simulink subsystem "adaptiveEcm"  (R2025b)
settings: Solver=VariableStepAuto  StartTime=0.0  StopTime=10.0  RelTol=1e-3
values from neighbouring files (symbols this model uses):
  ECM = ecmParams(TempDep=false, Degradation=false, IC=struct("soc0", zD(1, :), "T0C", mean(tC(1, :))))    [checkFastPlant.m]
undefined symbols (not defined in the file or in its folder): diff, trace
(part 2 of 2)

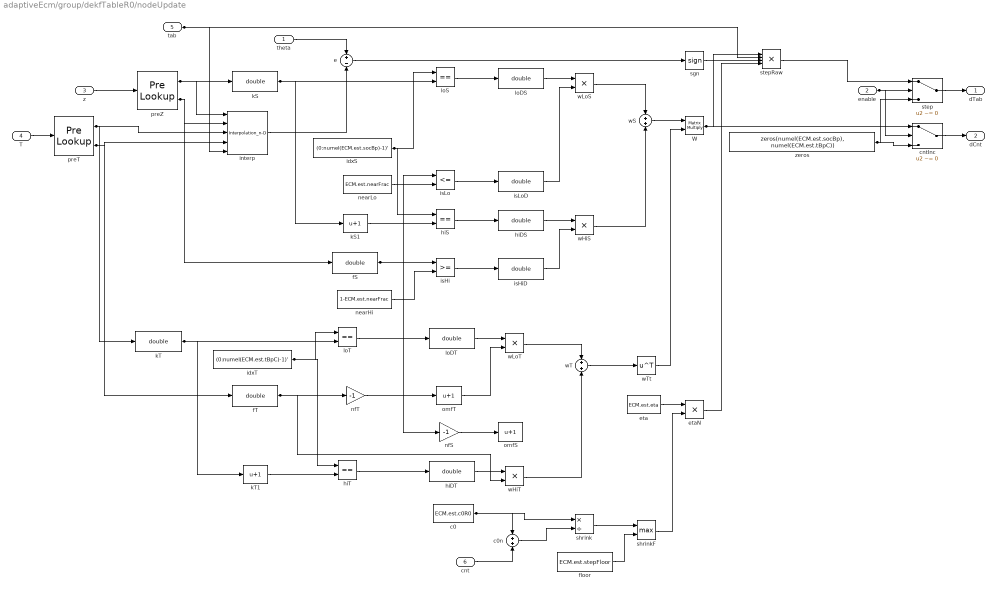
== system adaptiveEcm/group/dekfTableR0/nodeUpdate ==
  theta : Inport  PortDimensions=1
  enable : Inport  Port=2  PortDimensions=1
  z : Inport  Port=3  PortDimensions=1
  T : Inport  Port=4  PortDimensions=1
  tab : Inport  Port=5  PortDimensions=[numel(ECM.est.socBp) numel(ECM.est.tBpC)]
  cnt : Inport  Port=6  PortDimensions=[numel(ECM.est.socBp) numel(ECM.est.tBpC)]
  W : Product  Multiplication=Matrix(*)
  c0 : Constant  Value=ECM.est.c0R0
  c0n : Sum
  cntInc : Switch  Criteria=u2 ~= 0  SaturateOnIntegerOverflow=off  InputSameDT=off
  e : Sum  Inputs=+-
  eta : Constant  Value=ECM.est.eta
  etaN : Product
  fS : DataTypeConversion  OutDataTypeStr=double  SaturateOnIntegerOverflow=off  RndMeth=Floor
  fT : DataTypeConversion  OutDataTypeStr=double  SaturateOnIntegerOverflow=off  RndMeth=Floor
  floor : Constant  Value=ECM.est.stepFloor
  hiDS : DataTypeConversion  OutDataTypeStr=double  SaturateOnIntegerOverflow=off  RndMeth=Floor
  hiDT : DataTypeConversion  OutDataTypeStr=double  SaturateOnIntegerOverflow=off  RndMeth=Floor
  hiS : RelationalOperator  Operator===  OutDataTypeStr=boolean  RndMeth=Simplest  InputSameDT=off
  hiT : RelationalOperator  Operator===  OutDataTypeStr=boolean  RndMeth=Simplest  InputSameDT=off
  idxS : Constant  Value=(0:numel(ECM.est.socBp)-1)'
  idxT : Constant  Value=(0:numel(ECM.est.tBpC)-1)'
  interp : Interpolation_n-D  TableSource=Input port  InternalRulePriority=Speed
      settings: InputPortMap=u0,u1,u2,u3,p2
  isHi : RelationalOperator  OutDataTypeStr=boolean  RndMeth=Simplest  InputSameDT=off
  isHiD : DataTypeConversion  OutDataTypeStr=double  SaturateOnIntegerOverflow=off  RndMeth=Floor
  isLo : RelationalOperator  Operator=<=  OutDataTypeStr=boolean  RndMeth=Simplest  InputSameDT=off
  isLoD : DataTypeConversion  OutDataTypeStr=double  SaturateOnIntegerOverflow=off  RndMeth=Floor
  kS : DataTypeConversion  OutDataTypeStr=double  SaturateOnIntegerOverflow=off  RndMeth=Floor
  kS1 : Bias  Bias=1  SaturateOnIntegerOverflow=off
  kT : DataTypeConversion  OutDataTypeStr=double  SaturateOnIntegerOverflow=off  RndMeth=Floor
  kT1 : Bias  Bias=1  SaturateOnIntegerOverflow=off
  loDS : DataTypeConversion  OutDataTypeStr=double  SaturateOnIntegerOverflow=off  RndMeth=Floor
  loDT : DataTypeConversion  OutDataTypeStr=double  SaturateOnIntegerOverflow=off  RndMeth=Floor
  loS : RelationalOperator  Operator===  OutDataTypeStr=boolean  RndMeth=Simplest  InputSameDT=off
  loT : RelationalOperator  Operator===  OutDataTypeStr=boolean  RndMeth=Simplest  InputSameDT=off
  nearHi : Constant  Value=1-ECM.est.nearFrac
  nearLo : Constant  Value=ECM.est.nearFrac
  nfS : Gain  Gain=-1
  nfT : Gain  Gain=-1
  omfS : Bias  Bias=1  SaturateOnIntegerOverflow=off
  omfT : Bias  Bias=1  SaturateOnIntegerOverflow=off
  preT : PreLookup  BreakpointsData=ECM.est.tBpC
  preZ : PreLookup  BreakpointsData=ECM.est.socBp
  sgn : Signum
  shrink : Product  Inputs=*/
  shrinkF : MinMax  Function=max  Inputs=2
  step : Switch  Criteria=u2 ~= 0  SaturateOnIntegerOverflow=off  InputSameDT=off
  stepRaw : Product  Inputs=4
  wHiS : Product
  wHiT : Product
  wLoS : Product
  wLoT : Product
  wS : Sum
  wT : Sum
  wTt : Math  Operator=transpose
  zeros : Constant  Value=zeros(numel(ECM.est.socBp), numel(ECM.est.tBpC))
  dTab : Outport
  dCnt : Outport  Port=2
  wires:
  kT/1 -> loT/2, kT1/1
  T/1 -> preT/1
  zeros/1 -> cntInc/3, step/3
  hiT/1 -> hiDT/1
  nearHi/1 -> isHi/2
  kS1/1 -> hiS/2
  z/1 -> preZ/1
  preZ/1 -> interp/1, kS/1
  preT/1 -> interp/3, kT/1
  preZ/2 -> fS/1, interp/2
  tab/1 -> stepRaw/2, interp/5
  preT/2 -> interp/4, fT/1
  wLoS/1 -> wS/1
  c0/1 -> shrink/1, c0n/1
  loT/1 -> loDT/1
  theta/1 -> e/1
  wHiS/1 -> wS/2
  kS/1 -> loS/2, kS1/1
  isHi/1 -> isHiD/1
  interp/1 -> e/2
  cntInc/1 -> dCnt/1
  wLoT/1 -> wT/1
  idxT/1 -> loT/1, hiT/1
  fT/1 -> wHiT/2, nfT/1
  kT1/1 -> hiT/2
  e/1 -> sgn/1
  eta/1 -> etaN/1
  idxS/1 -> hiS/1, loS/1
  shrink/1 -> shrinkF/1
  nearLo/1 -> isLo/2
  loDS/1 -> wLoS/1
  fS/1 -> nfS/1, isLo/1, isHi/1
  nfT/1 -> omfT/1
  step/1 -> dTab/1
  enable/1 -> cntInc/2, step/2
  sgn/1 -> stepRaw/3
  loS/1 -> loDS/1
  isLo/1 -> isLoD/1
  isHiD/1 -> wHiS/2
  hiS/1 -> hiDS/1
  loDT/1 -> wLoT/1
  omfT/1 -> wLoT/2
  shrinkF/1 -> etaN/2
  nfS/1 -> omfS/1
  hiDT/1 -> wHiT/1
  cnt/1 -> c0n/2
  isLoD/1 -> wLoS/2
  W/1 -> cntInc/1, stepRaw/1
  hiDS/1 -> wHiS/1
  wHiT/1 -> wT/2
  c0n/1 -> shrink/2
  wT/1 -> wTt/1
  floor/1 -> shrinkF/2
  wS/1 -> W/1
  wTt/1 -> W/2
  etaN/1 -> stepRaw/4
  stepRaw/1 -> step/1

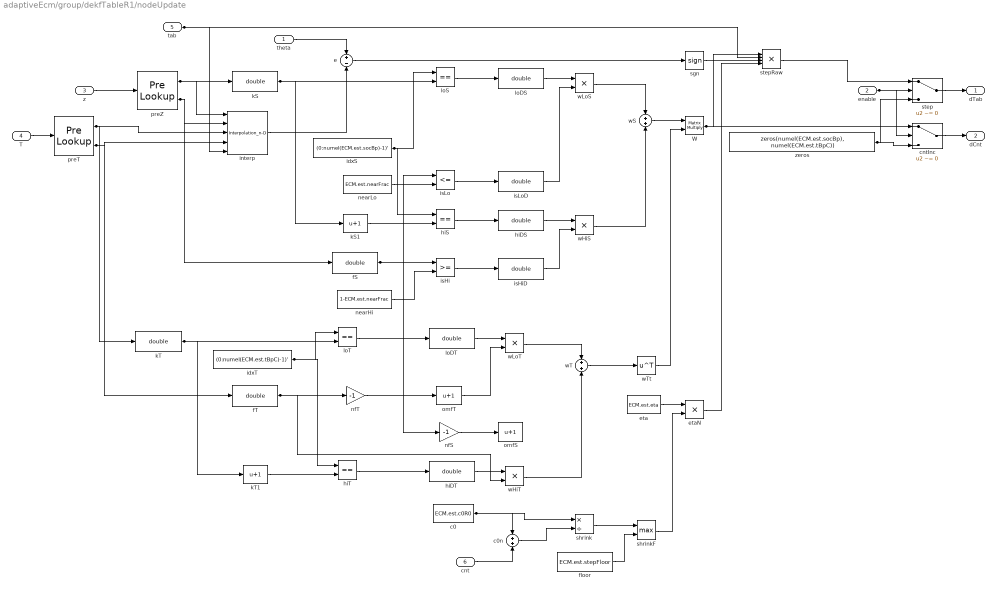
== system adaptiveEcm/group/dekfTableR1/nodeUpdate ==
  theta : Inport  PortDimensions=1
  enable : Inport  Port=2  PortDimensions=1
  z : Inport  Port=3  PortDimensions=1
  T : Inport  Port=4  PortDimensions=1
  tab : Inport  Port=5  PortDimensions=[numel(ECM.est.socBp) numel(ECM.est.tBpC)]
  cnt : Inport  Port=6  PortDimensions=[numel(ECM.est.socBp) numel(ECM.est.tBpC)]
  W : Product  Multiplication=Matrix(*)
  c0 : Constant  Value=ECM.est.c0R0
  c0n : Sum
  cntInc : Switch  Criteria=u2 ~= 0  SaturateOnIntegerOverflow=off  InputSameDT=off
  e : Sum  Inputs=+-
  eta : Constant  Value=ECM.est.eta
  etaN : Product
  fS : DataTypeConversion  OutDataTypeStr=double  SaturateOnIntegerOverflow=off  RndMeth=Floor
  fT : DataTypeConversion  OutDataTypeStr=double  SaturateOnIntegerOverflow=off  RndMeth=Floor
  floor : Constant  Value=ECM.est.stepFloor
  hiDS : DataTypeConversion  OutDataTypeStr=double  SaturateOnIntegerOverflow=off  RndMeth=Floor
  hiDT : DataTypeConversion  OutDataTypeStr=double  SaturateOnIntegerOverflow=off  RndMeth=Floor
  hiS : RelationalOperator  Operator===  OutDataTypeStr=boolean  RndMeth=Simplest  InputSameDT=off
  hiT : RelationalOperator  Operator===  OutDataTypeStr=boolean  RndMeth=Simplest  InputSameDT=off
  idxS : Constant  Value=(0:numel(ECM.est.socBp)-1)'
  idxT : Constant  Value=(0:numel(ECM.est.tBpC)-1)'
  interp : Interpolation_n-D  TableSource=Input port  InternalRulePriority=Speed
      settings: InputPortMap=u0,u1,u2,u3,p2
  isHi : RelationalOperator  OutDataTypeStr=boolean  RndMeth=Simplest  InputSameDT=off
  isHiD : DataTypeConversion  OutDataTypeStr=double  SaturateOnIntegerOverflow=off  RndMeth=Floor
  isLo : RelationalOperator  Operator=<=  OutDataTypeStr=boolean  RndMeth=Simplest  InputSameDT=off
  isLoD : DataTypeConversion  OutDataTypeStr=double  SaturateOnIntegerOverflow=off  RndMeth=Floor
  kS : DataTypeConversion  OutDataTypeStr=double  SaturateOnIntegerOverflow=off  RndMeth=Floor
  kS1 : Bias  Bias=1  SaturateOnIntegerOverflow=off
  kT : DataTypeConversion  OutDataTypeStr=double  SaturateOnIntegerOverflow=off  RndMeth=Floor
  kT1 : Bias  Bias=1  SaturateOnIntegerOverflow=off
  loDS : DataTypeConversion  OutDataTypeStr=double  SaturateOnIntegerOverflow=off  RndMeth=Floor
  loDT : DataTypeConversion  OutDataTypeStr=double  SaturateOnIntegerOverflow=off  RndMeth=Floor
  loS : RelationalOperator  Operator===  OutDataTypeStr=boolean  RndMeth=Simplest  InputSameDT=off
  loT : RelationalOperator  Operator===  OutDataTypeStr=boolean  RndMeth=Simplest  InputSameDT=off
  nearHi : Constant  Value=1-ECM.est.nearFrac
  nearLo : Constant  Value=ECM.est.nearFrac
  nfS : Gain  Gain=-1
  nfT : Gain  Gain=-1
  omfS : Bias  Bias=1  SaturateOnIntegerOverflow=off
  omfT : Bias  Bias=1  SaturateOnIntegerOverflow=off
  preT : PreLookup  BreakpointsData=ECM.est.tBpC
  preZ : PreLookup  BreakpointsData=ECM.est.socBp
  sgn : Signum
  shrink : Product  Inputs=*/
  shrinkF : MinMax  Function=max  Inputs=2
  step : Switch  Criteria=u2 ~= 0  SaturateOnIntegerOverflow=off  InputSameDT=off
  stepRaw : Product  Inputs=4
  wHiS : Product
  wHiT : Product
  wLoS : Product
  wLoT : Product
  wS : Sum
  wT : Sum
  wTt : Math  Operator=transpose
  zeros : Constant  Value=zeros(numel(ECM.est.socBp), numel(ECM.est.tBpC))
  dTab : Outport
  dCnt : Outport  Port=2
  wires:
  wT/1 -> wTt/1
  preZ/1 -> interp/1, kS/1
  step/1 -> dTab/1
  preT/1 -> interp/3, kT/1
  c0/1 -> shrink/1, c0n/1
  T/1 -> preT/1
  floor/1 -> shrinkF/2
  hiT/1 -> hiDT/1
  preZ/2 -> fS/1, interp/2
  cntInc/1 -> dCnt/1
  wLoT/1 -> wT/1
  z/1 -> preZ/1
  preT/2 -> interp/4, fT/1
  hiDT/1 -> wHiT/1
  tab/1 -> interp/5, stepRaw/2
  hiS/1 -> hiDS/1
  kT/1 -> loT/2, kT1/1
  wTt/1 -> W/2
  loDT/1 -> wLoT/1
  fT/1 -> wHiT/2, nfT/1
  theta/1 -> e/1
  kS/1 -> kS1/1, loS/2
  interp/1 -> e/2
  idxT/1 -> loT/1, hiT/1
  kT1/1 -> hiT/2
  idxS/1 -> loS/1, hiS/1
  e/1 -> sgn/1
  loT/1 -> loDT/1
  nearLo/1 -> isLo/2
  nearHi/1 -> isHi/2
  kS1/1 -> hiS/2
  loDS/1 -> wLoS/1
  fS/1 -> nfS/1, isLo/1, isHi/1
  nfT/1 -> omfT/1
  loS/1 -> loDS/1
  isLo/1 -> isLoD/1
  isHi/1 -> isHiD/1
  shrinkF/1 -> etaN/2
  omfT/1 -> wLoT/2
  nfS/1 -> omfS/1
  cnt/1 -> c0n/2
  isLoD/1 -> wLoS/2
  hiDS/1 -> wHiS/1
  isHiD/1 -> wHiS/2
  wHiT/1 -> wT/2
  c0n/1 -> shrink/2
  wLoS/1 -> wS/1
  wHiS/1 -> wS/2
  shrink/1 -> shrinkF/1
  wS/1 -> W/1
  eta/1 -> etaN/1
  sgn/1 -> stepRaw/3
  enable/1 -> step/2, cntInc/2
  W/1 -> cntInc/1, stepRaw/1
  etaN/1 -> stepRaw/4
  stepRaw/1 -> step/1
  zeros/1 -> step/3, cntInc/3

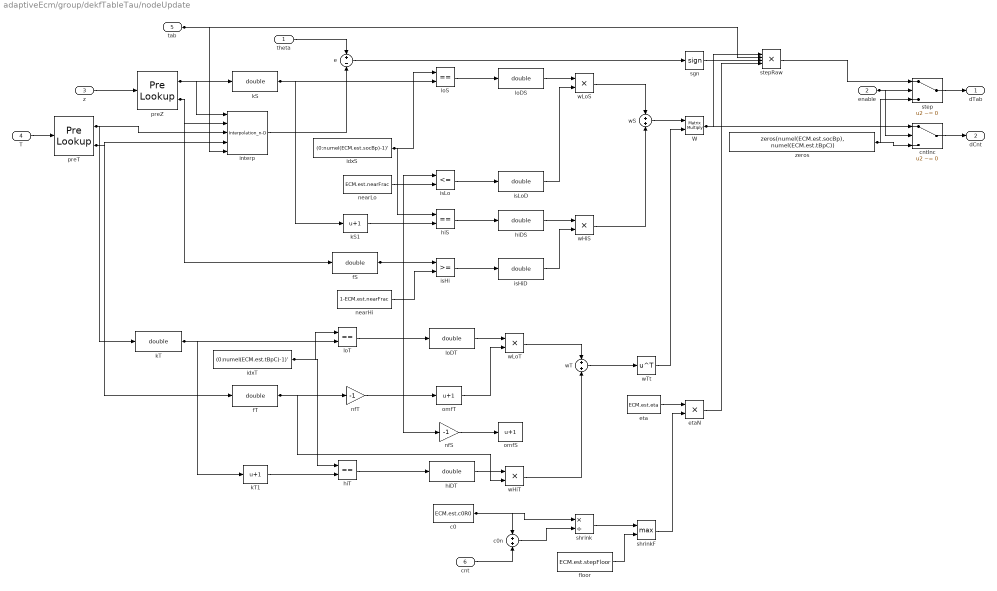
== system adaptiveEcm/group/dekfTableTau/nodeUpdate ==
  theta : Inport  PortDimensions=1
  enable : Inport  Port=2  PortDimensions=1
  z : Inport  Port=3  PortDimensions=1
  T : Inport  Port=4  PortDimensions=1
  tab : Inport  Port=5  PortDimensions=[numel(ECM.est.socBp) numel(ECM.est.tBpC)]
  cnt : Inport  Port=6  PortDimensions=[numel(ECM.est.socBp) numel(ECM.est.tBpC)]
  W : Product  Multiplication=Matrix(*)
  c0 : Constant  Value=ECM.est.c0R0
  c0n : Sum
  cntInc : Switch  Criteria=u2 ~= 0  SaturateOnIntegerOverflow=off  InputSameDT=off
  e : Sum  Inputs=+-
  eta : Constant  Value=ECM.est.eta
  etaN : Product
  fS : DataTypeConversion  OutDataTypeStr=double  SaturateOnIntegerOverflow=off  RndMeth=Floor
  fT : DataTypeConversion  OutDataTypeStr=double  SaturateOnIntegerOverflow=off  RndMeth=Floor
  floor : Constant  Value=ECM.est.stepFloor
  hiDS : DataTypeConversion  OutDataTypeStr=double  SaturateOnIntegerOverflow=off  RndMeth=Floor
  hiDT : DataTypeConversion  OutDataTypeStr=double  SaturateOnIntegerOverflow=off  RndMeth=Floor
  hiS : RelationalOperator  Operator===  OutDataTypeStr=boolean  RndMeth=Simplest  InputSameDT=off
  hiT : RelationalOperator  Operator===  OutDataTypeStr=boolean  RndMeth=Simplest  InputSameDT=off
  idxS : Constant  Value=(0:numel(ECM.est.socBp)-1)'
  idxT : Constant  Value=(0:numel(ECM.est.tBpC)-1)'
  interp : Interpolation_n-D  TableSource=Input port  InternalRulePriority=Speed
      settings: InputPortMap=u0,u1,u2,u3,p2
  isHi : RelationalOperator  OutDataTypeStr=boolean  RndMeth=Simplest  InputSameDT=off
  isHiD : DataTypeConversion  OutDataTypeStr=double  SaturateOnIntegerOverflow=off  RndMeth=Floor
  isLo : RelationalOperator  Operator=<=  OutDataTypeStr=boolean  RndMeth=Simplest  InputSameDT=off
  isLoD : DataTypeConversion  OutDataTypeStr=double  SaturateOnIntegerOverflow=off  RndMeth=Floor
  kS : DataTypeConversion  OutDataTypeStr=double  SaturateOnIntegerOverflow=off  RndMeth=Floor
  kS1 : Bias  Bias=1  SaturateOnIntegerOverflow=off
  kT : DataTypeConversion  OutDataTypeStr=double  SaturateOnIntegerOverflow=off  RndMeth=Floor
  kT1 : Bias  Bias=1  SaturateOnIntegerOverflow=off
  loDS : DataTypeConversion  OutDataTypeStr=double  SaturateOnIntegerOverflow=off  RndMeth=Floor
  loDT : DataTypeConversion  OutDataTypeStr=double  SaturateOnIntegerOverflow=off  RndMeth=Floor
  loS : RelationalOperator  Operator===  OutDataTypeStr=boolean  RndMeth=Simplest  InputSameDT=off
  loT : RelationalOperator  Operator===  OutDataTypeStr=boolean  RndMeth=Simplest  InputSameDT=off
  nearHi : Constant  Value=1-ECM.est.nearFrac
  nearLo : Constant  Value=ECM.est.nearFrac
  nfS : Gain  Gain=-1
  nfT : Gain  Gain=-1
  omfS : Bias  Bias=1  SaturateOnIntegerOverflow=off
  omfT : Bias  Bias=1  SaturateOnIntegerOverflow=off
  preT : PreLookup  BreakpointsData=ECM.est.tBpC
  preZ : PreLookup  BreakpointsData=ECM.est.socBp
  sgn : Signum
  shrink : Product  Inputs=*/
  shrinkF : MinMax  Function=max  Inputs=2
  step : Switch  Criteria=u2 ~= 0  SaturateOnIntegerOverflow=off  InputSameDT=off
  stepRaw : Product  Inputs=4
  wHiS : Product
  wHiT : Product
  wLoS : Product
  wLoT : Product
  wS : Sum
  wT : Sum
  wTt : Math  Operator=transpose
  zeros : Constant  Value=zeros(numel(ECM.est.socBp), numel(ECM.est.tBpC))
  dTab : Outport
  dCnt : Outport  Port=2
  wires:
  hiS/1 -> hiDS/1
  preZ/1 -> interp/1, kS/1
  kS1/1 -> hiS/2
  preT/1 -> interp/3, kT/1
  c0n/1 -> shrink/2
  T/1 -> preT/1
  fT/1 -> wHiT/2, nfT/1
  z/1 -> preZ/1
  cntInc/1 -> dCnt/1
  wLoT/1 -> wT/1
  preZ/2 -> fS/1, interp/2
  hiT/1 -> hiDT/1
  preT/2 -> interp/4, fT/1
  isHi/1 -> isHiD/1
  tab/1 -> stepRaw/2, interp/5
  wT/1 -> wTt/1
  kT/1 -> loT/2, kT1/1
  loS/1 -> loDS/1
  idxS/1 -> loS/1, hiS/1
  theta/1 -> e/1
  kS/1 -> loS/2, kS1/1
  interp/1 -> e/2
  idxT/1 -> loT/1, hiT/1
  stepRaw/1 -> step/1
  kT1/1 -> hiT/2
  wHiT/1 -> wT/2
  e/1 -> sgn/1
  nearLo/1 -> isLo/2
  fS/1 -> nfS/1, isLo/1, isHi/1
  nearHi/1 -> isHi/2
  loT/1 -> loDT/1
  nfT/1 -> omfT/1
  isLo/1 -> isLoD/1
  loDT/1 -> wLoT/1
  omfT/1 -> wLoT/2
  zeros/1 -> cntInc/3, step/3
  nfS/1 -> omfS/1
  hiDT/1 -> wHiT/1
  c0/1 -> shrink/1, c0n/1
  W/1 -> stepRaw/1, cntInc/1
  loDS/1 -> wLoS/1
  cnt/1 -> c0n/2
  step/1 -> dTab/1
  isLoD/1 -> wLoS/2
  hiDS/1 -> wHiS/1
  enable/1 -> cntInc/2, step/2
  isHiD/1 -> wHiS/2
  wLoS/1 -> wS/1
  wHiS/1 -> wS/2
  shrink/1 -> shrinkF/1
  floor/1 -> shrinkF/2
  wS/1 -> W/1
  wTt/1 -> W/2
  eta/1 -> etaN/1
  shrinkF/1 -> etaN/2
  sgn/1 -> stepRaw/3
  etaN/1 -> stepRaw/4

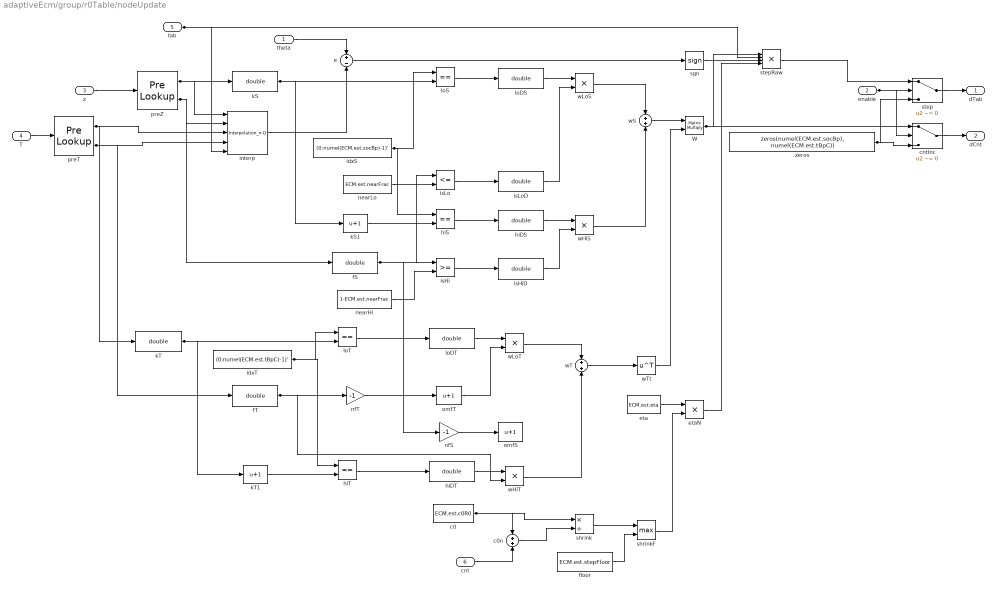
== system adaptiveEcm/group/r0Table/nodeUpdate ==
  theta : Inport  PortDimensions=1
  enable : Inport  Port=2  PortDimensions=1
  z : Inport  Port=3  PortDimensions=1
  T : Inport  Port=4  PortDimensions=1
  tab : Inport  Port=5  PortDimensions=[numel(ECM.est.socBp) numel(ECM.est.tBpC)]
  cnt : Inport  Port=6  PortDimensions=[numel(ECM.est.socBp) numel(ECM.est.tBpC)]
  W : Product  Multiplication=Matrix(*)
  c0 : Constant  Value=ECM.est.c0R0
  c0n : Sum
  cntInc : Switch  Criteria=u2 ~= 0  SaturateOnIntegerOverflow=off  InputSameDT=off
  e : Sum  Inputs=+-
  eta : Constant  Value=ECM.est.eta
  etaN : Product
  fS : DataTypeConversion  OutDataTypeStr=double  SaturateOnIntegerOverflow=off  RndMeth=Floor
  fT : DataTypeConversion  OutDataTypeStr=double  SaturateOnIntegerOverflow=off  RndMeth=Floor
  floor : Constant  Value=ECM.est.stepFloor
  hiDS : DataTypeConversion  OutDataTypeStr=double  SaturateOnIntegerOverflow=off  RndMeth=Floor
  hiDT : DataTypeConversion  OutDataTypeStr=double  SaturateOnIntegerOverflow=off  RndMeth=Floor
  hiS : RelationalOperator  Operator===  OutDataTypeStr=boolean  RndMeth=Simplest  InputSameDT=off
  hiT : RelationalOperator  Operator===  OutDataTypeStr=boolean  RndMeth=Simplest  InputSameDT=off
  idxS : Constant  Value=(0:numel(ECM.est.socBp)-1)'
  idxT : Constant  Value=(0:numel(ECM.est.tBpC)-1)'
  interp : Interpolation_n-D  TableSource=Input port  InternalRulePriority=Speed
      settings: InputPortMap=u0,u1,u2,u3,p2
  isHi : RelationalOperator  OutDataTypeStr=boolean  RndMeth=Simplest  InputSameDT=off
  isHiD : DataTypeConversion  OutDataTypeStr=double  SaturateOnIntegerOverflow=off  RndMeth=Floor
  isLo : RelationalOperator  Operator=<=  OutDataTypeStr=boolean  RndMeth=Simplest  InputSameDT=off
  isLoD : DataTypeConversion  OutDataTypeStr=double  SaturateOnIntegerOverflow=off  RndMeth=Floor
  kS : DataTypeConversion  OutDataTypeStr=double  SaturateOnIntegerOverflow=off  RndMeth=Floor
  kS1 : Bias  Bias=1  SaturateOnIntegerOverflow=off
  kT : DataTypeConversion  OutDataTypeStr=double  SaturateOnIntegerOverflow=off  RndMeth=Floor
  kT1 : Bias  Bias=1  SaturateOnIntegerOverflow=off
  loDS : DataTypeConversion  OutDataTypeStr=double  SaturateOnIntegerOverflow=off  RndMeth=Floor
  loDT : DataTypeConversion  OutDataTypeStr=double  SaturateOnIntegerOverflow=off  RndMeth=Floor
  loS : RelationalOperator  Operator===  OutDataTypeStr=boolean  RndMeth=Simplest  InputSameDT=off
  loT : RelationalOperator  Operator===  OutDataTypeStr=boolean  RndMeth=Simplest  InputSameDT=off
  nearHi : Constant  Value=1-ECM.est.nearFrac
  nearLo : Constant  Value=ECM.est.nearFrac
  nfS : Gain  Gain=-1
  nfT : Gain  Gain=-1
  omfS : Bias  Bias=1  SaturateOnIntegerOverflow=off
  omfT : Bias  Bias=1  SaturateOnIntegerOverflow=off
  preT : PreLookup  BreakpointsData=ECM.est.tBpC
  preZ : PreLookup  BreakpointsData=ECM.est.socBp
  sgn : Signum
  shrink : Product  Inputs=*/
  shrinkF : MinMax  Function=max  Inputs=2
  step : Switch  Criteria=u2 ~= 0  SaturateOnIntegerOverflow=off  InputSameDT=off
  stepRaw : Product  Inputs=4
  wHiS : Product
  wHiT : Product
  wLoS : Product
  wLoT : Product
  wS : Sum
  wT : Sum
  wTt : Math  Operator=transpose
  zeros : Constant  Value=zeros(numel(ECM.est.socBp), numel(ECM.est.tBpC))
  dTab : Outport
  dCnt : Outport  Port=2
  wires:
  preZ/2 -> fS/1, interp/2
  isLoD/1 -> wLoS/2
  T/1 -> preT/1
  wTt/1 -> W/2
  isHiD/1 -> wHiS/2
  loDT/1 -> wLoT/1
  fT/1 -> wHiT/2, nfT/1
  kT/1 -> kT1/1, loT/2
  preT/2 -> interp/4, fT/1
  z/1 -> preZ/1
  tab/1 -> stepRaw/2, interp/5
  preT/1 -> interp/3, kT/1
  omfT/1 -> wLoT/2
  preZ/1 -> interp/1, kS/1
  cntInc/1 -> dCnt/1
  fS/1 -> nfS/1, isLo/1, isHi/1
  theta/1 -> e/1
  c0n/1 -> shrink/2
  kT1/1 -> hiT/2
  kS/1 -> kS1/1, loS/2
  interp/1 -> e/2
  idxT/1 -> loT/1, hiT/1
  wLoT/1 -> wT/1
  idxS/1 -> loS/1, hiS/1
  e/1 -> sgn/1
  nearLo/1 -> isLo/2
  kS1/1 -> hiS/2
  nearHi/1 -> isHi/2
  loT/1 -> loDT/1
  hiS/1 -> hiDS/1
  isLo/1 -> isLoD/1
  nfT/1 -> omfT/1
  loDS/1 -> wLoS/1
  hiT/1 -> hiDT/1
  c0/1 -> c0n/1, shrink/1
  loS/1 -> loDS/1
  isHi/1 -> isHiD/1
  nfS/1 -> omfS/1
  hiDT/1 -> wHiT/1
  cnt/1 -> c0n/2
  floor/1 -> shrinkF/2
  hiDS/1 -> wHiS/1
  wHiT/1 -> wT/2
  step/1 -> dTab/1
  wLoS/1 -> wS/1
  wHiS/1 -> wS/2
  wT/1 -> wTt/1
  shrink/1 -> shrinkF/1
  wS/1 -> W/1
  eta/1 -> etaN/1
  shrinkF/1 -> etaN/2
  sgn/1 -> stepRaw/3
  W/1 -> cntInc/1, stepRaw/1
  etaN/1 -> stepRaw/4
  stepRaw/1 -> step/1
  enable/1 -> cntInc/2, step/2
  zeros/1 -> cntInc/3, step/3

== system adaptiveEcm/group/rcIdent/r1Table ==
  theta : Inport  PortDimensions=1
  enable : Inport  Port=2  PortDimensions=1
  z : Inport  Port=3  PortDimensions=1
  T : Inport  Port=4  PortDimensions=1
  first : Inport  Port=5  PortDimensions=1
  tab : Inport  Port=6  PortDimensions=[numel(ECM.est.socBp) numel(ECM.est.tBpC)]
  cnt : Inport  Port=7  PortDimensions=[numel(ECM.est.socBp) numel(ECM.est.tBpC)]
  TLag : Sum
  TLagA : Gain  Gain=ECM.est.lambdaRc
  TLagB : Gain  Gain=1-ECM.est.lambdaRc
  TLagMem : UnitDelay  SampleTime=-1  HasFrameUpgradeWarning=on
  TLagOld : Switch  Criteria=u2 > Threshold  Threshold=0.5  SaturateOnIntegerOverflow=off  InputSameDT=off
  nodeUpdate : Subsystem
  zLag : Sum
  zLagA : Gain  Gain=ECM.est.lambdaRc
  zLagB : Gain  Gain=1-ECM.est.lambdaRc
  zLagMem : UnitDelay  SampleTime=-1  HasFrameUpgradeWarning=on
  zLagOld : Switch  Criteria=u2 > Threshold  Threshold=0.5  SaturateOnIntegerOverflow=off  InputSameDT=off
  dTab : Outport
  dCnt : Outport  Port=2
  wires:
  z/1 -> zLagB/1, zLagOld/1
  zLagB/1 -> zLag/2
  TLagOld/1 -> TLagA/1
  first/1 -> zLagOld/2, TLagOld/2
  zLagOld/1 -> zLagA/1
  T/1 -> TLagOld/1, TLagB/1
  TLagB/1 -> TLag/2
  zLagA/1 -> zLag/1
  TLagA/1 -> TLag/1
  theta/1 -> nodeUpdate/1(theta)
  zLag/1 -> zLagMem/1, nodeUpdate/3(z)
  enable/1 -> nodeUpdate/2(enable)
  tab/1 -> nodeUpdate/5(tab)
  TLag/1 -> TLagMem/1, nodeUpdate/4(T)
  cnt/1 -> nodeUpdate/6(cnt)
  zLagMem/1 -> zLagOld/3
  nodeUpdate/1(dTab) -> dTab/1
  nodeUpdate/2(dCnt) -> dCnt/1
  TLagMem/1 -> TLagOld/3

== system adaptiveEcm/group/rcIdent/tauTable ==
  theta : Inport  PortDimensions=1
  enable : Inport  Port=2  PortDimensions=1
  z : Inport  Port=3  PortDimensions=1
  T : Inport  Port=4  PortDimensions=1
  first : Inport  Port=5  PortDimensions=1
  tab : Inport  Port=6  PortDimensions=[numel(ECM.est.socBp) numel(ECM.est.tBpC)]
  cnt : Inport  Port=7  PortDimensions=[numel(ECM.est.socBp) numel(ECM.est.tBpC)]
  TLag : Sum
  TLagA : Gain  Gain=ECM.est.lambdaRc
  TLagB : Gain  Gain=1-ECM.est.lambdaRc
  TLagMem : UnitDelay  SampleTime=-1  HasFrameUpgradeWarning=on
  TLagOld : Switch  Criteria=u2 > Threshold  Threshold=0.5  SaturateOnIntegerOverflow=off  InputSameDT=off
  nodeUpdate : Subsystem
  zLag : Sum
  zLagA : Gain  Gain=ECM.est.lambdaRc
  zLagB : Gain  Gain=1-ECM.est.lambdaRc
  zLagMem : UnitDelay  SampleTime=-1  HasFrameUpgradeWarning=on
  zLagOld : Switch  Criteria=u2 > Threshold  Threshold=0.5  SaturateOnIntegerOverflow=off  InputSameDT=off
  dTab : Outport
  dCnt : Outport  Port=2
  wires:
  theta/1 -> nodeUpdate/1(theta)
  z/1 -> zLagB/1, zLagOld/1
  first/1 -> zLagOld/2, TLagOld/2
  zLagOld/1 -> zLagA/1
  TLagOld/1 -> TLagA/1
  T/1 -> TLagOld/1, TLagB/1
  TLagB/1 -> TLag/2
  zLagA/1 -> zLag/1
  zLagB/1 -> zLag/2
  TLagA/1 -> TLag/1
  zLag/1 -> zLagMem/1, nodeUpdate/3(z)
  enable/1 -> nodeUpdate/2(enable)
  tab/1 -> nodeUpdate/5(tab)
  TLag/1 -> TLagMem/1, nodeUpdate/4(T)
  cnt/1 -> nodeUpdate/6(cnt)
  zLagMem/1 -> zLagOld/3
  nodeUpdate/1(dTab) -> dTab/1
  nodeUpdate/2(dCnt) -> dCnt/1
  TLagMem/1 -> TLagOld/3

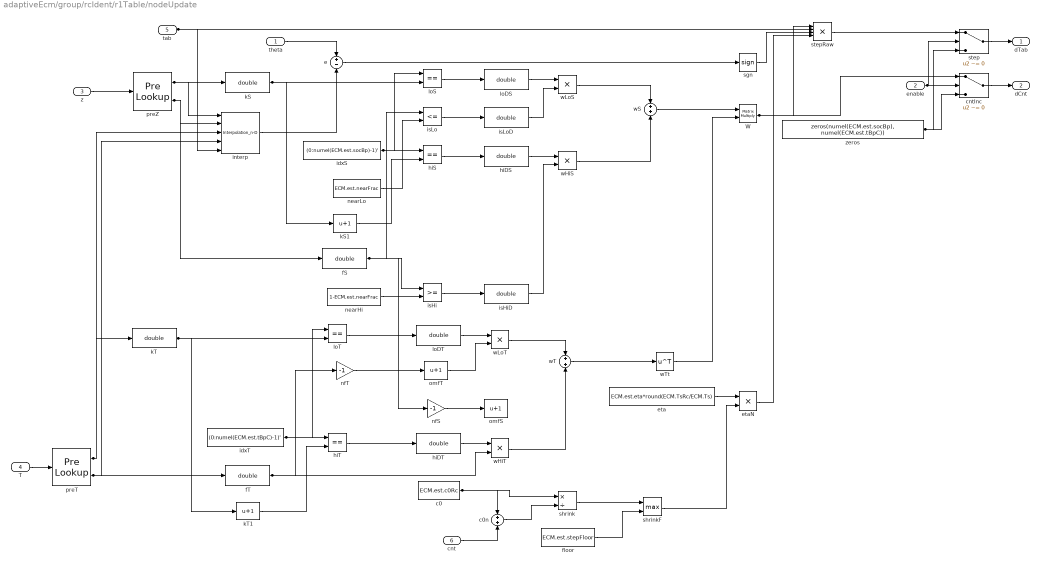
== system adaptiveEcm/group/rcIdent/r1Table/nodeUpdate ==
  theta : Inport  PortDimensions=1
  enable : Inport  Port=2  PortDimensions=1
  z : Inport  Port=3  PortDimensions=1
  T : Inport  Port=4  PortDimensions=1
  tab : Inport  Port=5  PortDimensions=[numel(ECM.est.socBp) numel(ECM.est.tBpC)]
  cnt : Inport  Port=6  PortDimensions=[numel(ECM.est.socBp) numel(ECM.est.tBpC)]
  W : Product  Multiplication=Matrix(*)
  c0 : Constant  Value=ECM.est.c0Rc
  c0n : Sum
  cntInc : Switch  Criteria=u2 ~= 0  SaturateOnIntegerOverflow=off  InputSameDT=off
  e : Sum  Inputs=+-
  eta : Constant  Value=ECM.est.eta*round(ECM.TsRc/ECM.Ts)
  etaN : Product
  fS : DataTypeConversion  OutDataTypeStr=double  SaturateOnIntegerOverflow=off  RndMeth=Floor
  fT : DataTypeConversion  OutDataTypeStr=double  SaturateOnIntegerOverflow=off  RndMeth=Floor
  floor : Constant  Value=ECM.est.stepFloor
  hiDS : DataTypeConversion  OutDataTypeStr=double  SaturateOnIntegerOverflow=off  RndMeth=Floor
  hiDT : DataTypeConversion  OutDataTypeStr=double  SaturateOnIntegerOverflow=off  RndMeth=Floor
  hiS : RelationalOperator  Operator===  OutDataTypeStr=boolean  RndMeth=Simplest  InputSameDT=off
  hiT : RelationalOperator  Operator===  OutDataTypeStr=boolean  RndMeth=Simplest  InputSameDT=off
  idxS : Constant  Value=(0:numel(ECM.est.socBp)-1)'
  idxT : Constant  Value=(0:numel(ECM.est.tBpC)-1)'
  interp : Interpolation_n-D  TableSource=Input port  InternalRulePriority=Speed
      settings: InputPortMap=u0,u1,u2,u3,p2
  isHi : RelationalOperator  OutDataTypeStr=boolean  RndMeth=Simplest  InputSameDT=off
  isHiD : DataTypeConversion  OutDataTypeStr=double  SaturateOnIntegerOverflow=off  RndMeth=Floor
  isLo : RelationalOperator  Operator=<=  OutDataTypeStr=boolean  RndMeth=Simplest  InputSameDT=off
  isLoD : DataTypeConversion  OutDataTypeStr=double  SaturateOnIntegerOverflow=off  RndMeth=Floor
  kS : DataTypeConversion  OutDataTypeStr=double  SaturateOnIntegerOverflow=off  RndMeth=Floor
  kS1 : Bias  Bias=1  SaturateOnIntegerOverflow=off
  kT : DataTypeConversion  OutDataTypeStr=double  SaturateOnIntegerOverflow=off  RndMeth=Floor
  kT1 : Bias  Bias=1  SaturateOnIntegerOverflow=off
  loDS : DataTypeConversion  OutDataTypeStr=double  SaturateOnIntegerOverflow=off  RndMeth=Floor
  loDT : DataTypeConversion  OutDataTypeStr=double  SaturateOnIntegerOverflow=off  RndMeth=Floor
  loS : RelationalOperator  Operator===  OutDataTypeStr=boolean  RndMeth=Simplest  InputSameDT=off
  loT : RelationalOperator  Operator===  OutDataTypeStr=boolean  RndMeth=Simplest  InputSameDT=off
  nearHi : Constant  Value=1-ECM.est.nearFrac
  nearLo : Constant  Value=ECM.est.nearFrac
  nfS : Gain  Gain=-1
  nfT : Gain  Gain=-1
  omfS : Bias  Bias=1  SaturateOnIntegerOverflow=off
  omfT : Bias  Bias=1  SaturateOnIntegerOverflow=off
  preT : PreLookup  BreakpointsData=ECM.est.tBpC
  preZ : PreLookup  BreakpointsData=ECM.est.socBp
  sgn : Signum
  shrink : Product  Inputs=*/
  shrinkF : MinMax  Function=max  Inputs=2
  step : Switch  Criteria=u2 ~= 0  SaturateOnIntegerOverflow=off  InputSameDT=off
  stepRaw : Product  Inputs=4
  wHiS : Product
  wHiT : Product
  wLoS : Product
  wLoT : Product
  wS : Sum
  wT : Sum
  wTt : Math  Operator=transpose
  zeros : Constant  Value=zeros(numel(ECM.est.socBp), numel(ECM.est.tBpC))
  dTab : Outport
  dCnt : Outport  Port=2
  wires:
  sgn/1 -> stepRaw/3
  T/1 -> preT/1
  preZ/2 -> fS/1, interp/2
  isHi/1 -> isHiD/1
  fT/1 -> wHiT/2, nfT/1
  preZ/1 -> interp/1, kS/1
  z/1 -> preZ/1
  eta/1 -> etaN/1
  kT/1 -> kT1/1, loT/2
  preT/1 -> interp/3, kT/1
  preT/2 -> interp/4, fT/1
  tab/1 -> stepRaw/2, interp/5
  theta/1 -> e/1
  cntInc/1 -> dCnt/1
  kS/1 -> loS/2, kS1/1
  wHiT/1 -> wT/2
  interp/1 -> e/2
  nearHi/1 -> isHi/2
  e/1 -> sgn/1
  idxT/1 -> loT/1, hiT/1
  kT1/1 -> hiT/2
  idxS/1 -> loS/1, hiS/1
  hiDT/1 -> wHiT/1
  nearLo/1 -> isLo/2
  W/1 -> cntInc/1, stepRaw/1
  kS1/1 -> hiS/2
  fS/1 -> nfS/1, isLo/1, isHi/1
  wHiS/1 -> wS/2
  loT/1 -> loDT/1
  nfT/1 -> omfT/1
  hiS/1 -> hiDS/1
  hiT/1 -> hiDT/1
  isHiD/1 -> wHiS/2
  loS/1 -> loDS/1
  isLo/1 -> isLoD/1
  loDT/1 -> wLoT/1
  shrinkF/1 -> etaN/2
  omfT/1 -> wLoT/2
  step/1 -> dTab/1
  nfS/1 -> omfS/1
  c0/1 -> shrink/1, c0n/1
  cnt/1 -> c0n/2
  wTt/1 -> W/2
  loDS/1 -> wLoS/1
  isLoD/1 -> wLoS/2
  etaN/1 -> stepRaw/4
  wT/1 -> wTt/1
  hiDS/1 -> wHiS/1
  wLoT/1 -> wT/1
  c0n/1 -> shrink/2
  wLoS/1 -> wS/1
  shrink/1 -> shrinkF/1
  floor/1 -> shrinkF/2
  wS/1 -> W/1
  stepRaw/1 -> step/1
  enable/1 -> cntInc/2, step/2
  zeros/1 -> cntInc/3, step/3

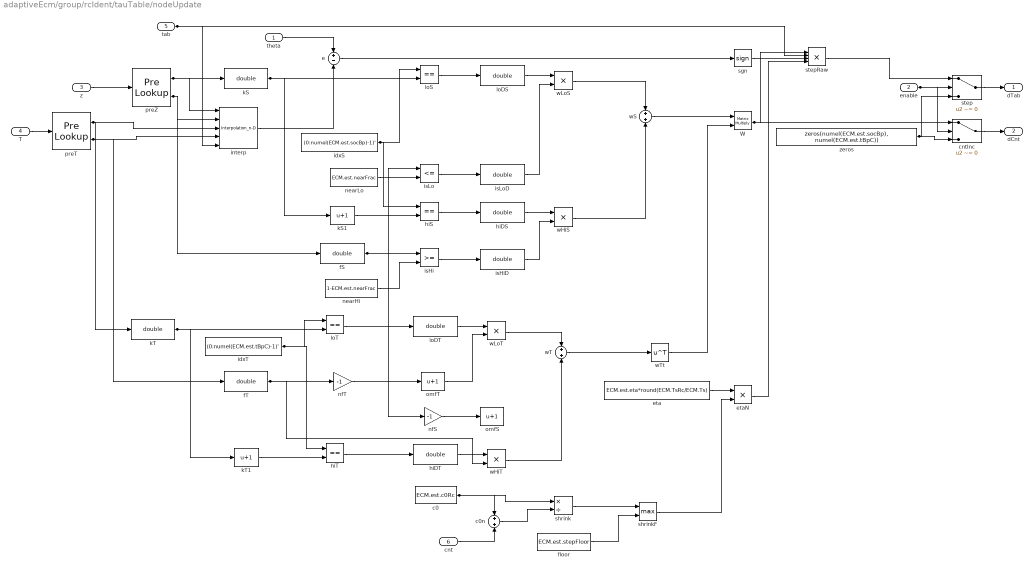
== system adaptiveEcm/group/rcIdent/tauTable/nodeUpdate ==
  theta : Inport  PortDimensions=1
  enable : Inport  Port=2  PortDimensions=1
  z : Inport  Port=3  PortDimensions=1
  T : Inport  Port=4  PortDimensions=1
  tab : Inport  Port=5  PortDimensions=[numel(ECM.est.socBp) numel(ECM.est.tBpC)]
  cnt : Inport  Port=6  PortDimensions=[numel(ECM.est.socBp) numel(ECM.est.tBpC)]
  W : Product  Multiplication=Matrix(*)
  c0 : Constant  Value=ECM.est.c0Rc
  c0n : Sum
  cntInc : Switch  Criteria=u2 ~= 0  SaturateOnIntegerOverflow=off  InputSameDT=off
  e : Sum  Inputs=+-
  eta : Constant  Value=ECM.est.eta*round(ECM.TsRc/ECM.Ts)
  etaN : Product
  fS : DataTypeConversion  OutDataTypeStr=double  SaturateOnIntegerOverflow=off  RndMeth=Floor
  fT : DataTypeConversion  OutDataTypeStr=double  SaturateOnIntegerOverflow=off  RndMeth=Floor
  floor : Constant  Value=ECM.est.stepFloor
  hiDS : DataTypeConversion  OutDataTypeStr=double  SaturateOnIntegerOverflow=off  RndMeth=Floor
  hiDT : DataTypeConversion  OutDataTypeStr=double  SaturateOnIntegerOverflow=off  RndMeth=Floor
  hiS : RelationalOperator  Operator===  OutDataTypeStr=boolean  RndMeth=Simplest  InputSameDT=off
  hiT : RelationalOperator  Operator===  OutDataTypeStr=boolean  RndMeth=Simplest  InputSameDT=off
  idxS : Constant  Value=(0:numel(ECM.est.socBp)-1)'
  idxT : Constant  Value=(0:numel(ECM.est.tBpC)-1)'
  interp : Interpolation_n-D  TableSource=Input port  InternalRulePriority=Speed
      settings: InputPortMap=u0,u1,u2,u3,p2
  isHi : RelationalOperator  OutDataTypeStr=boolean  RndMeth=Simplest  InputSameDT=off
  isHiD : DataTypeConversion  OutDataTypeStr=double  SaturateOnIntegerOverflow=off  RndMeth=Floor
  isLo : RelationalOperator  Operator=<=  OutDataTypeStr=boolean  RndMeth=Simplest  InputSameDT=off
  isLoD : DataTypeConversion  OutDataTypeStr=double  SaturateOnIntegerOverflow=off  RndMeth=Floor
  kS : DataTypeConversion  OutDataTypeStr=double  SaturateOnIntegerOverflow=off  RndMeth=Floor
  kS1 : Bias  Bias=1  SaturateOnIntegerOverflow=off
  kT : DataTypeConversion  OutDataTypeStr=double  SaturateOnIntegerOverflow=off  RndMeth=Floor
  kT1 : Bias  Bias=1  SaturateOnIntegerOverflow=off
  loDS : DataTypeConversion  OutDataTypeStr=double  SaturateOnIntegerOverflow=off  RndMeth=Floor
  loDT : DataTypeConversion  OutDataTypeStr=double  SaturateOnIntegerOverflow=off  RndMeth=Floor
  loS : RelationalOperator  Operator===  OutDataTypeStr=boolean  RndMeth=Simplest  InputSameDT=off
  loT : RelationalOperator  Operator===  OutDataTypeStr=boolean  RndMeth=Simplest  InputSameDT=off
  nearHi : Constant  Value=1-ECM.est.nearFrac
  nearLo : Constant  Value=ECM.est.nearFrac
  nfS : Gain  Gain=-1
  nfT : Gain  Gain=-1
  omfS : Bias  Bias=1  SaturateOnIntegerOverflow=off
  omfT : Bias  Bias=1  SaturateOnIntegerOverflow=off
  preT : PreLookup  BreakpointsData=ECM.est.tBpC
  preZ : PreLookup  BreakpointsData=ECM.est.socBp
  sgn : Signum
  shrink : Product  Inputs=*/
  shrinkF : MinMax  Function=max  Inputs=2
  step : Switch  Criteria=u2 ~= 0  SaturateOnIntegerOverflow=off  InputSameDT=off
  stepRaw : Product  Inputs=4
  wHiS : Product
  wHiT : Product
  wLoS : Product
  wLoT : Product
  wS : Sum
  wT : Sum
  wTt : Math  Operator=transpose
  zeros : Constant  Value=zeros(numel(ECM.est.socBp), numel(ECM.est.tBpC))
  dTab : Outport
  dCnt : Outport  Port=2
  wires:
  cntInc/1 -> dCnt/1
  preZ/1 -> interp/1, kS/1
  stepRaw/1 -> step/1
  T/1 -> preT/1
  z/1 -> preZ/1
  sgn/1 -> stepRaw/3
  preT/2 -> interp/4, fT/1
  preT/1 -> interp/3, kT/1
  kT/1 -> loT/2, kT1/1
  tab/1 -> interp/5, stepRaw/2
  W/1 -> cntInc/1, stepRaw/1
  shrink/1 -> shrinkF/1
  nfS/1 -> omfS/1
  preZ/2 -> fS/1, interp/2
  nearHi/1 -> isHi/2
  theta/1 -> e/1
  wT/1 -> wTt/1
  isHi/1 -> isHiD/1
  kS/1 -> loS/2, kS1/1
  interp/1 -> e/2
  idxT/1 -> loT/1, hiT/1
  loDT/1 -> wLoT/1
  hiS/1 -> hiDS/1
  fT/1 -> nfT/1, wHiT/2
  wLoT/1 -> wT/1
  kT1/1 -> hiT/2
  e/1 -> sgn/1
  cnt/1 -> c0n/2
  idxS/1 -> loS/1, hiS/1
  nearLo/1 -> isLo/2
  wHiS/1 -> wS/2
  kS1/1 -> hiS/2
  fS/1 -> isLo/1, nfS/1, isHi/1
  isHiD/1 -> wHiS/2
  loT/1 -> loDT/1
  nfT/1 -> omfT/1
  hiT/1 -> hiDT/1
  loS/1 -> loDS/1
  isLo/1 -> isLoD/1
  omfT/1 -> wLoT/2
  hiDT/1 -> wHiT/1
  c0/1 -> c0n/1, shrink/1
  loDS/1 -> wLoS/1
  isLoD/1 -> wLoS/2
  hiDS/1 -> wHiS/1
  enable/1 -> step/2, cntInc/2
  wHiT/1 -> wT/2
  c0n/1 -> shrink/2
  zeros/1 -> cntInc/3, step/3
  eta/1 -> etaN/1
  wLoS/1 -> wS/1
  floor/1 -> shrinkF/2
  wS/1 -> W/1
  wTt/1 -> W/2
  shrinkF/1 -> etaN/2
  etaN/1 -> stepRaw/4
  step/1 -> dTab/1
